simulink model "with_Arduin"  (R2017a)
settings: Solver=VariableStepAuto  StartTime=0.0  StopTime=inf  MaxStep=1e-4  RelTol=1e-3
libraries: powerlib x10, arduino_io_lib x5
settings Model: Creator=Ahmed  LastModifiedBy=Ahmed

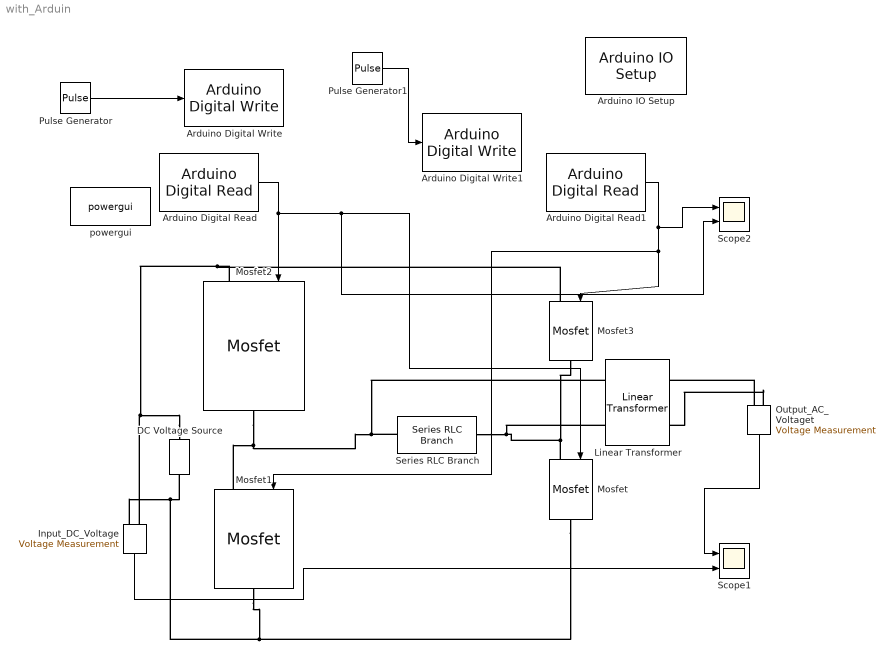
== system with_Arduin ==
  Arduino Digital Read : arduino_io_lib/Arduino Digital Read  arduinoVar=Temporary arduino variable: Arduino1  arduinoPin=9  T=0.01
  Arduino Digital Read1 : arduino_io_lib/Arduino Digital Read  arduinoVar=Temporary arduino variable: Arduino1  arduinoPin=10  T=0.01
  Arduino Digital Write : arduino_io_lib/Arduino Digital Write  arduinoVar=Temporary arduino variable: Arduino1  arduinoPin=4  T=0.01
  Arduino Digital Write1 : arduino_io_lib/Arduino Digital Write  arduinoVar=Temporary arduino variable: Arduino1  arduinoPin=5  T=0.01
  Arduino IO Setup : arduino_io_lib/Arduino IO Setup  Priority=3  arduinoVar=Temporary arduino variable: Arduino1  workspaceVarName=a  comPort=COM5
  DC Voltage Source : powerlib/Electrical Sources/DC Voltage Source  Amplitude=12  Measurements=None
  Input_DC_Voltage : powerlib/Measurements/Voltage Measurement  PhasorSimulation=off  OutputType=Complex  PSBequivalent=0
  Linear Transformer : powerlib/Elements/Linear Transformer  UNITS=SI  NominalPower=[75e3,60]  winding1=[12 0 0]  winding2=[220 0 0]  ThreeWindings=off  winding3=[3.15e+05 315.06 0.088675]  RmLm=[Inf Inf]  Measurements=Winding voltages  DataType=on
  Mosfet{,1..3} (4 alike) : powerlib/Power Electronics/Mosfet  Ron=0.1  Lon=0  Rd=0.01  Vfd=0  IC=0  Rs=1e5  Cs=inf  Measurements=off
  Output_AC_Voltaget : powerlib/Measurements/Voltage Measurement  PhasorSimulation=off  OutputType=Complex  PSBequivalent=0
  Pulse Generator : DiscretePulseGenerator  PulseType=Time based  Period=0.02  PulseWidth=50
  Pulse Generator1 : DiscretePulseGenerator  PulseType=Time based  Period=0.02  PulseWidth=50  PhaseDelay=0.01
  Scope1 : Scope  NumInputPorts=2
  Scope2 : Scope  NumInputPorts=2
  Series RLC Branch : powerlib/Elements/Series RLC Branch  LConnTagsString=__new0  RConnTagsString=__new0  BranchType=R  Resistance=5  Inductance=1e-3  SetiL0=off  InitialCurrent=0  Capacitance=1e-6  Setx0=off  InitialVoltage=0  Measurements=None
  powergui : powerlib/powergui  Priority=1  SimulationMode=Continuous  SampleTime=50e-6  frequency=60  Iterations=50  frequencyindice=0  Pbase=100e6  ErrMax=1e-4  UnitsV=kV  UnitsW=MW  buscounter=0  FunctionMessages=off  echomessages=off  EnableUseOfTLC=off  CurrentSourceSwitches=off  DisableSnubberDevices=off  DisableRonSwitches=off  DisableVfSwitches=off  DisplayEquations=off  SolverType=Tustin/Backward Euler (TBE)  Interpol=off  ExternalGateDelay=off  methode=off  Ts=100  x0status=blocks  SPID=on  SwTol=0  HookPort=off  RestoreLinks=warning  ResistiveCurrentMeasurement=off  Frange=[0:2:500]  Ylog=off  Xlog=on  ShowGrid=off  save=off  variable=ZData  structure=0  ZoomFFT=off  StartTime=0.0  cycles=1  DisplayStyle=1  fundamental=60  FreqAxis=off  MaxFrequency=1000  frequencyindicesteady=1  RmsSteady=1  display=off
  wires:
  Output_AC_Voltaget/1 -> Scope1/1
  Pulse Generator/1 -> Arduino Digital Write/1
  Pulse Generator1/1 -> Arduino Digital Write1/1
  Arduino Digital Read/1 -> Scope2/2, Mosfet/1, Mosfet2/1
  Arduino Digital Read1/1 -> Scope2/1, Mosfet1/1, Mosfet3/1
  Input_DC_Voltage/1 -> Scope1/2
  connections:
  Linear Transformer/LConn2 -- Series RLC Branch/RConn1 -- Mosfet/LConn1 -- Mosfet3/RConn1
  Linear Transformer/LConn1 -- Series RLC Branch/LConn1 -- Mosfet1/LConn1 -- Mosfet2/RConn1
  DC Voltage Source/RConn1 -- Input_DC_Voltage/LConn1 -- Mosfet3/LConn1 -- Mosfet2/LConn1
  DC Voltage Source/LConn1 -- Input_DC_Voltage/LConn2 -- Mosfet1/RConn1 -- Mosfet/RConn1
  Output_AC_Voltaget/LConn2 -- Linear Transformer/RConn1
  Output_AC_Voltaget/LConn1 -- Linear Transformer/RConn2
